simulink model "simulacionsimulink"  (R2026a)
settings: Solver=VariableStepAuto  StopTime=5
settings Model: Creator=molin  LastModifiedBy=molin

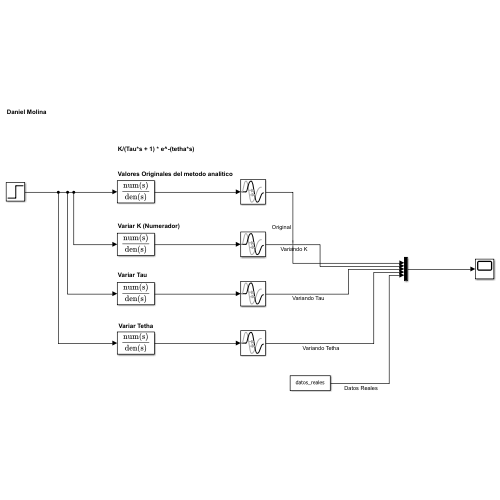
[thumbnail: Simulink's stored preview of the top-level diagram]
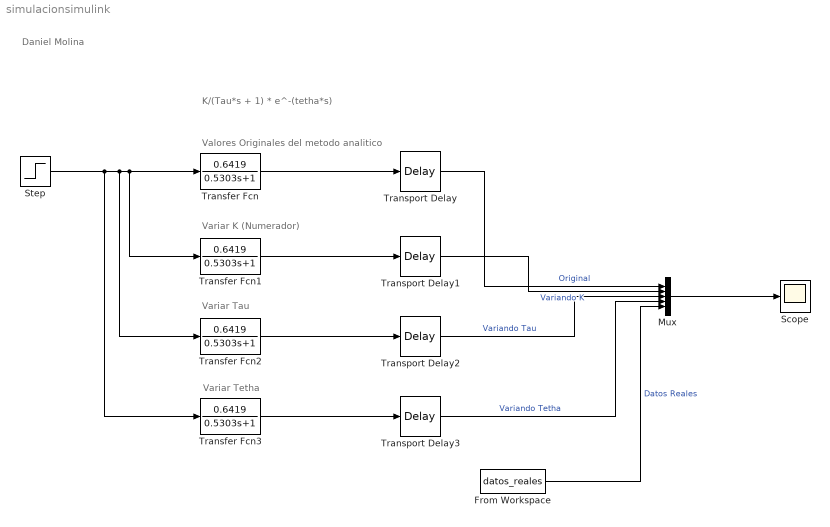
== system simulacionsimulink ==
  note: Valores Originales del metodo analitico
  note: Variar K (Numerador)
  note: Variar Tau
  note: Variar Tetha
  note: K/(Tau*s + 1) * e^-(tetha*s)
  note: Daniel Molina
  From Workspace : FromWorkspace  VariableName=datos_reales
  Mux : Mux  Inputs=5
  Scope : Scope
      settings: ActiveDisplayYMinimum=-0.091308621900901721  ActiveDisplayYMaximum=1.3664172911091454
  Step : Step  Time=0.25  FinalValue=1.5  SampleTime=0
  Transfer Fcn{,1..3} (4 alike) : TransferFcn  Numerator=[0.6419]  Denominator=[0.5303 1]
  Transport Delay : TransportDelay  DelayTime=0.1768
  Transport Delay1 : TransportDelay  DelayTime=0.1768
  Transport Delay2 : TransportDelay  DelayTime=0.1768
  Transport Delay3 : TransportDelay  DelayTime=0.5
  wires:
  Step/1 -> Transfer Fcn3/1, Transfer Fcn2/1, Transfer Fcn1/1, Transfer Fcn/1
  Transfer Fcn/1 -> Transport Delay/1
  Mux/1 -> Scope/1
  Transfer Fcn1/1 -> Transport Delay1/1
  Transfer Fcn2/1 -> Transport Delay2/1
  Transfer Fcn3/1 -> Transport Delay3/1
  Transport Delay/1 -> Mux/1  "Original"
  Transport Delay1/1 -> Mux/2  "Variando K"
  Transport Delay2/1 -> Mux/3  "Variando Tau"
  Transport Delay3/1 -> Mux/4  "Variando Tetha"
  From Workspace/1 -> Mux/5  "Datos Reales"
